simulink model "arm2r_pd_gravity"  (R2024b)
settings: Solver=ode4  StartTime=0.0  StopTime=5  FixedStep=0.001  RelTol=1e-3
undefined symbols (not defined in the file): dq0, gc, Kd, Kp, q0, qref, tau_max
settings Model: Creator=ENVY  LastModifiedBy=ENVY

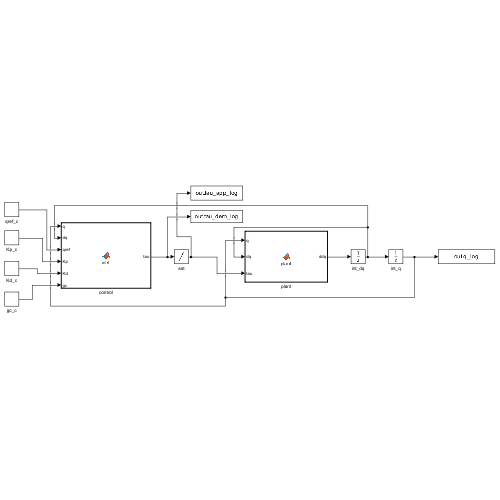
[thumbnail: Simulink's stored preview of the top-level diagram]
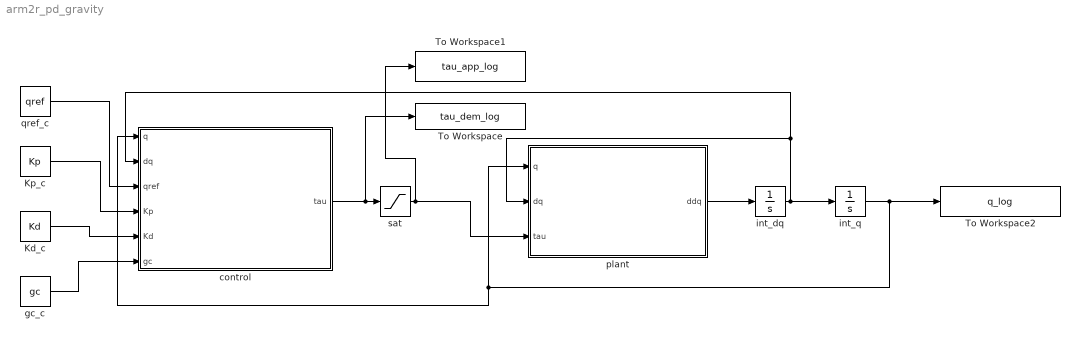
== system arm2r_pd_gravity ==
  Kd_c : Constant  Value=Kd
  Kp_c : Constant  Value=Kp
  To Workspace : ToWorkspace  VariableName=tau_dem_log  SampleTime=-1
      settings: Save2DSignal=2-D array (concatenate along first dimension)
  To Workspace1 : ToWorkspace  VariableName=tau_app_log  SampleTime=-1
      settings: Save2DSignal=2-D array (concatenate along first dimension)
  To Workspace2 : ToWorkspace  VariableName=q_log  SampleTime=-1
      settings: Save2DSignal=2-D array (concatenate along first dimension)
  control : MATLAB Function  TreatAsAtomicUnit=on
  gc_c : Constant  Value=gc
  int_dq : Integrator  InitialCondition=dq0
  int_q : Integrator  InitialCondition=q0
  plant : MATLAB Function  TreatAsAtomicUnit=on
  qref_c : Constant  Value=qref
  sat : Saturate  UpperLimit=tau_max  LowerLimit=-tau_max
  wires:
  qref_c/1 -> control/3(qref)
  Kp_c/1 -> control/4(Kp)
  Kd_c/1 -> control/5(Kd)
  gc_c/1 -> control/6(gc)
  control/1(tau) -> To Workspace/1, sat/1
  sat/1 -> To Workspace1/1, plant/3(tau)
  plant/1(ddq) -> int_dq/1
  int_dq/1 -> control/2(dq), plant/2(dq), int_q/1
  int_q/1 -> To Workspace2/1, plant/1(q), control/1(q)

== matlab function arm2r_pd_gravity/plant ==
  data: q input; ddq output; dq input; tau input
function ddq = plant(q, dq, tau)

q   = q(:);
dq  = dq(:);
tau = tau(:);

ddq = arm2rDynamics(q, dq, tau);
ddq = ddq(:);
end

== matlab function arm2r_pd_gravity/control ==
  data: q input; tau output; dq input; qref input; Kp input; Kd input; gc input
function tau = ctrl(q, dq, qref, Kp, Kd, gc)
%CTRL Control law A: PD + optional gravity compensation.

q    = q(:);      % force column vector, whatever came in
dq   = dq(:);
qref = qref(:);

tau = arm2rPdGravity(q, dq, qref, Kp, Kd, gc);
tau = tau(:);     % force column output
end
